simulink model "comparison_simulation"  (R2026b)
settings: Solver=VariableStepAuto  StopTime=1
InitFcn:
  | run param_file.m
values from neighbouring files (symbols this model uses):
  param = struct()    [param_file.m]
settings Model: Creator=mahmu  LastModifiedBy=mahmu

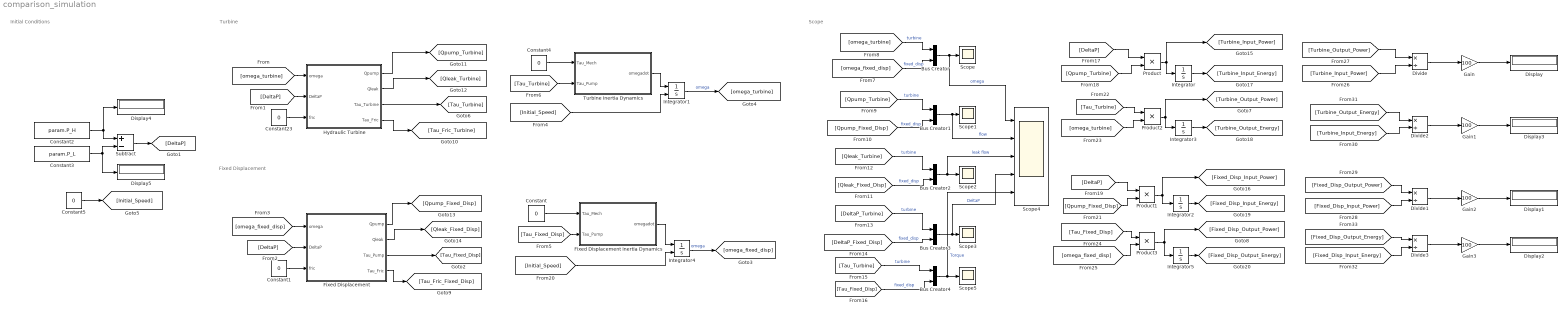
== system comparison_simulation ==
  note: Scope
  note: Fixed Displacement
  note: Turbine
  note: Initial Conditions
  Bus Creator{,1..4} (5 alike) : BusCreator  Inputs=2
  Constant{,1,4..5,23} (5 alike) : Constant  Value=0
  Constant2 : Constant  Value=param.P_H
  Constant3 : Constant  Value=param.P_L
  Display{,1..5} (6 alike) : Display
  Divide{,1..3} (4 alike) : Product  Inputs=*/
  Fixed Displacement : MATLAB Function  TreatAsAtomicUnit=on
  Fixed Displacement Inertia Dynamics : MATLAB Function  TreatAsAtomicUnit=on
  Gain{,1..3} (4 alike) : Gain  Gain=100
  Hydraulic Turbine : MATLAB Function  TreatAsAtomicUnit=on
  Integrator{,2..3,5} (4 alike) : Integrator
  Integrator1 : Integrator  InitialConditionSource=external
  Integrator4 : Integrator  InitialConditionSource=external
  Product{,1..3} (4 alike) : Product
  Scope{,1..3,5} (5 alike) : Scope
      Scope settings: ActiveDisplayYMinimum=-365.79111087287282  ActiveDisplayYMaximum=3292.1199978558561
      Scope1 settings: ActiveDisplayYMinimum=-4.2811547892902191E-5  ActiveDisplayYMaximum=0.00042292815958304392
      Scope2 settings: DataLoggingVariableName=ScopeData2
      Scope3 settings: ActiveDisplayYMinimum=5.895E+6  ActiveDisplayYMaximum=7.895E+6  DataLoggingVariableName=ScopeData3
      Scope5 settings: ActiveDisplayYMinimum=-0.0010343154987941228  ActiveDisplayYMaximum=0.0093088394891471075  DataLoggingVariableName=ScopeData5
  Scope4 : Scope  NumInputPorts=5
      settings: ActiveDisplayYMinimum=-543.28468228253143  ActiveDisplayYMaximum=4889.5621405427837  DataLoggingVariableName=ScopeData4
  Subtract : Sum  Inputs=+-
  Turbine Inertia Dynamics : MATLAB Function  TreatAsAtomicUnit=on
  wires:
  Hydraulic Turbine/1(Qpump) -> [Qpump_Turbine]
  Constant23/1 -> Hydraulic Turbine/3(fric)
  Hydraulic Turbine/4(Tau_Fric) -> [Tau_Fric_Turbine]
  [omega_turbine] -> Hydraulic Turbine/1(omega)
  Hydraulic Turbine/2(Qleak) -> [Qleak_Turbine]
  Hydraulic Turbine/3(Tau_Turbine) -> [Tau_Turbine]
  Fixed Displacement/1(Qpump) -> [Qpump_Fixed_Disp]
  [omega_fixed_disp] -> Fixed Displacement/1(omega)
  Constant1/1 -> Fixed Displacement/3(fric)
  Fixed Displacement/4(Tau_Fric) -> [Tau_Fric_Fixed_Disp]
  Fixed Displacement/2(Qleak) -> [Qleak_Fixed_Disp]
  Fixed Displacement/3(Tau_Pump) -> [Tau_Fixed_Disp]
  [Initial_Speed] -> Integrator4/2
  Constant/1 -> Fixed Displacement Inertia Dynamics/1(Tau_Mech)
  Fixed Displacement Inertia Dynamics/1(omegadot) -> Integrator4/1
  [Tau_Fixed_Disp] -> Fixed Displacement Inertia Dynamics/2(Tau_Pump)
  Integrator4/1 -> [omega_fixed_disp]  "omega"
  Constant2/1 -> Subtract/1, Display4/1
  Constant3/1 -> Subtract/2, Display5/1
  Integrator1/1 -> [omega_turbine]  "omega"
  [Tau_Turbine] -> Turbine Inertia Dynamics/2(Tau_Pump)
  Turbine Inertia Dynamics/1(omegadot) -> Integrator1/1
  Constant4/1 -> Turbine Inertia Dynamics/1(Tau_Mech)
  [Initial_Speed] -> Integrator1/2
  Constant5/1 -> [Initial_Speed]
  [omega_fixed_disp] -> Bus Creator/2  "fixed_disp"
  [omega_turbine] -> Bus Creator/1  "turbine"
  Bus Creator/1 -> Scope4/1, Scope/1  "omega"
  Bus Creator1/1 -> Scope4/2, Scope1/1  "flow"
  [Qpump_Turbine] -> Bus Creator1/1  "turbine"
  [Qpump_Fixed_Disp] -> Bus Creator1/2  "fixed_disp"
  [Qleak_Fixed_Disp] -> Bus Creator2/2  "fixed_disp"
  Bus Creator2/1 -> Scope4/3, Scope2/1  "leak flow"
  Bus Creator3/1 -> Scope4/4, Scope3/1  "DeltaP"
  [DeltaP_Turbine] -> Bus Creator3/1  "turbine"
  [DeltaP_Fixed_Disp] -> Bus Creator3/2  "fixed_disp"
  [Qleak_Turbine] -> Bus Creator2/1  "turbine"
  [Tau_Turbine] -> Bus Creator4/1  "turbine"
  [Tau_Fixed_Disp] -> Bus Creator4/2  "fixed_disp"
  Bus Creator4/1 -> Scope4/5, Scope5/1  "Torque"
  [DeltaP] -> Product/1
  [Qpump_Turbine] -> Product/2
  Product/1 -> [Turbine_Input_Power], Integrator/1
  Product1/1 -> [Fixed_Disp_Input_Power], Integrator2/1
  [Qpump_Fixed_Disp] -> Product1/2
  [DeltaP] -> Product1/1
  Subtract/1 -> [DeltaP]
  [DeltaP] -> Hydraulic Turbine/2(DeltaP)
  [DeltaP] -> Fixed Displacement/2(DeltaP)
  [omega_turbine] -> Product2/2
  [Tau_Turbine] -> Product2/1
  Product2/1 -> [Turbine_Output_Power], Integrator3/1
  Product3/1 -> Integrator5/1, [Fixed_Disp_Output_Power]
  [Tau_Fixed_Disp] -> Product3/1
  [omega_fixed_disp] -> Product3/2
  Integrator/1 -> [Turbine_Input_Energy]
  Integrator3/1 -> [Turbine_Output_Energy]
  Integrator2/1 -> [Fixed_Disp_Input_Energy]
  Integrator5/1 -> [Fixed_Disp_Output_Energy]
  Divide/1 -> Gain/1
  Divide1/1 -> Gain2/1
  Divide3/1 -> Gain3/1
  Divide2/1 -> Gain1/1
  Gain/1 -> Display/1
  Gain1/1 -> Display3/1
  Gain2/1 -> Display1/1
  Gain3/1 -> Display2/1
  [Turbine_Output_Power] -> Divide/1
  [Turbine_Input_Power] -> Divide/2
  [Turbine_Output_Energy] -> Divide2/1
  [Turbine_Input_Energy] -> Divide2/2
  [Fixed_Disp_Output_Power] -> Divide1/1
  [Fixed_Disp_Input_Power] -> Divide1/2
  [Fixed_Disp_Output_Energy] -> Divide3/1
  [Fixed_Disp_Input_Energy] -> Divide3/2

== matlab function comparison_simulation/Fixed Displacement ==
  data: Qpump output; Qleak output; omega input; DeltaP input; fric input; param parameter; Tau_Pump output; Tau_Fric output
function [Qpump, Qleak, Tau_Pump, Tau_Fric] = Fixed_Disp(omega, DeltaP, fric, param)

    Tau_Ideal = (param.D/(2*pi)) * DeltaP;
    
    % Pump friction model
    if fric == 1
        Tau_fr_nom = ((1 - param.eta_m_nom)/param.eta_m_nom) ...
                      * (param.D/(2*pi)) * param.dp_nom;
        
        k = (Tau_fr_nom - param.tau0) / param.dp_nom;
        
        omega_nom_rad = 2*pi*param.omega_nom/60;
        
        s = tanh(4*omega/(5e-5*omega_nom_rad));
        
        Tau_Fric = (param.tau0 + k*abs(DeltaP)) * s;
    else
        Tau_Fric = 0;
    end

    Tau_Pump = Tau_Ideal - Tau_Fric;

    % Analytical leakage model (Simscape-equivalent)
    
    % Parameters
    D     = param.D;          
    eta_v = param.eta_v_nom;  % nominal volumetric efficiency
    omega_nom = param.omega_nom;      % [rad/s]
    DeltaP_nom = param.dp_nom;    % [Pa]
    rho   = param.rho;        % [kg/m^3]
    
    % Hagen–Poiseuille coefficient
    K = (D/(2*pi))*omega_nom*(1 - eta_v)/DeltaP_nom;
    
    % Mass leakage flow
    m_dot_leak = K * rho * DeltaP;
    
    % Convert to volumetric leakage
    Qleak = m_dot_leak / rho;
    
    % Ideal displacement flow
    Qideal = (D/(2*pi)) * omega;
    
    % Net flow (same convention as Simscape)
    Qpump = Qideal + Qleak;
end

== matlab function comparison_simulation/Turbine Inertia Dynamics ==
  data: Tau_Mech input; Tau_Pump input; omegadot output; param parameter
function omegadot  = Inertia_Dyn(Tau_Mech, Tau_Pump, param)

omegadot = (Tau_Pump + Tau_Mech) / (param.J_hyd);

end

== matlab function comparison_simulation/Hydraulic Turbine ==
  data: Qpump output; Qleak output; omega input; DeltaP input; fric input; param parameter; Tau_Turbine output; Tau_Fric output
function [Qpump, Qleak, Tau_Turbine, Tau_Fric] = ...
    Turbine(omega, DeltaP, fric, param)


% Turbine geometry (SI units)
rho  = param.rho;          % Oil density [kg/m^3]
r    = param.turb_r;       % Outlet moment arm [m]
Ain  = param.turb_Ain;     % Axial inlet flow area [m^2]
Aout = param.turb_Aout;    % Outlet flow area [m^2]

assert(rho > 0 && r > 0, ...
    'Turbine density and radius must be positive.');
assert(Ain > Aout && Aout > 0, ...
    'This turbine model requires Ain > Aout > 0.');

% Pressure-flow relationship: paper Eq. (14).
% Forward-flow branch only; do not extrapolate to reverse flow.
denominator = 1/Aout^2 - 1/Ain^2;
numerator   = 2*DeltaP/rho + (r*omega)^2;

assert(numerator >= 0, ...
    'Operating point is outside the forward-flow turbine model.');

Qpump = sqrt(numerator/denominator);

% Fluid-generated turbine torque: paper Eq. (15)
Tau_Ideal = rho*r*Qpump*(Qpump/Aout - r*omega);

% Optional viscous turbine/spool friction
if fric == 1
    Tau_Fric = param.turb_B * omega;
else
    Tau_Fric = 0;
end

% Net torque supplied to the existing inertia block
Tau_Turbine = Tau_Ideal - Tau_Fric;

% No separate leakage model in this turbine formulation
Qleak = 0;

end

== matlab function comparison_simulation/Fixed Displacement Inertia Dynamics ==
  data: Tau_Mech input; Tau_Pump input; omegadot output; param parameter
function omegadot  = Inertia_Dyn(Tau_Mech, Tau_Pump, param)

omegadot = (Tau_Pump + Tau_Mech) / (param.J_hyd);

end
